simulink model "Parallel_Inverter_VSG"  (R2021b)
settings: Solver=FixedStepAuto  StartTime=0.0  StopTime=1  RelTol=1e-3
libraries: spsSeriesRLCBranchLib x11, spsCurrentMeasurementLib x4, spsVoltageMeasurementLib x4, spsDCVoltageSourceLib x2, powerlib_extras x2, spsTHDLib x2, spsUniversalBridgeLib x2, simulink x2, spspowerguiLib x1
settings Model: SimulationMode=accelerator  Creator=abc6820292  LastModifiedBy=abc6820292
settings SolverCC: ZeroCrossControl=EnableAll  ZeroCrossAlgorithm=Adaptive
settings SFSimCC: SimTargetLang=C++
settings RTWCC: BuildConfiguration=Faster Runs

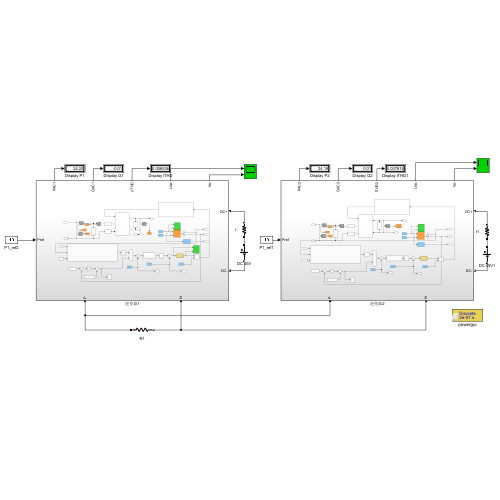
[thumbnail: Simulink's stored preview of the top-level diagram]
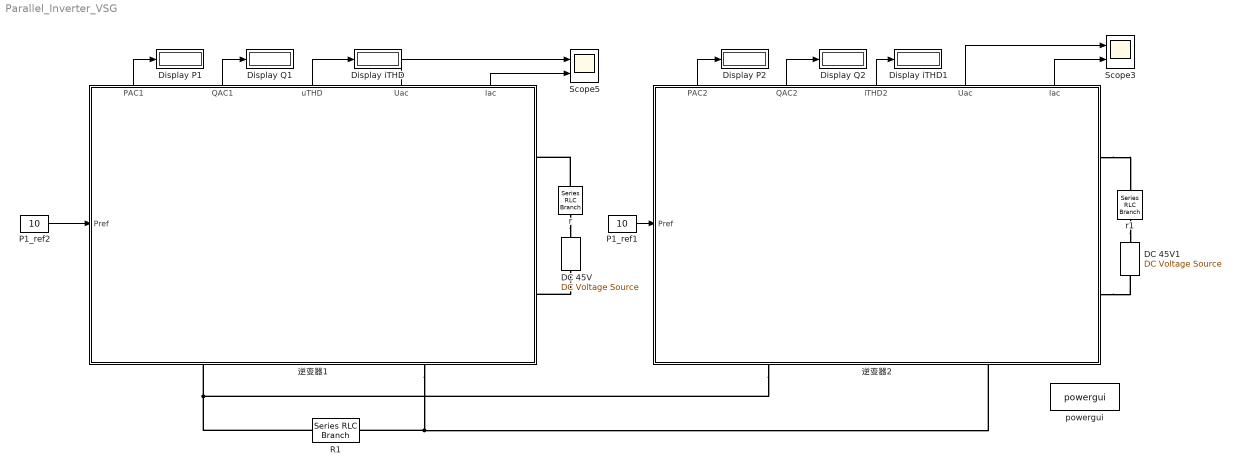
== system Parallel_Inverter_VSG ==
  DC 45V : spsDCVoltageSourceLib/DC Voltage Source  Amplitude=45  Measurements=None
  DC 45V1 : spsDCVoltageSourceLib/DC Voltage Source  Amplitude=45  Measurements=None
  Display P1 : Display
      settings: Format=bank
  Display P2 : Display
      settings: Format=bank
  Display Q1 : Display
      settings: Format=bank
  Display Q2 : Display
      settings: Format=bank
  Display iTHD : Display
  Display iTHD1 : Display
  P1_ref1 : Constant  Value=10
  P1_ref2 : Constant  Value=10
  R1 : spsSeriesRLCBranchLib/Series RLC Branch  LConnTagsString=__new0  RConnTagsString=__new0  BranchType=R  Resistance=12  Inductance=0  SetiL0=off  InitialCurrent=0  Capacitance=3e-4  Setx0=off  InitialVoltage=350  Measurements=None
  Scope3 : Scope  NumInputPorts=2
  Scope5 : Scope  NumInputPorts=2
  powergui : spspowerguiLib/powergui  SimulationMode=Discrete  SampleTime=2e-7  frequency=60  Iterations=50  frequencyindice=0  Pbase=100e6  ErrMax=1e-4  UnitsV=kV  UnitsW=MW  buscounter=0  FunctionMessages=off  echomessages=off  EnableUseOfTLC=off  CurrentSourceSwitches=off  DisableSnubberDevices=off  DisableRonSwitches=off  DisableVfSwitches=off  DisplayEquations=off  AutomaticDiscreteSolvers=off  SolverType=Tustin/Backward Euler (TBE)  Interpol=off  ExternalGateDelay=off  methode=off  Ts=0  x0status=blocks  SPID=off  SwTol=0  HookPort=off  NonlinearTolerance=1e-4  nMaxIteration=100  ContinueOnMaxIteration=off  RestoreLinks=warning  ResistiveCurrentMeasurement=off  Frange=[0:2:500]  Ylog=off  Xlog=on  ShowGrid=off  save=off  variable=ZData  structure=QQQQQ  ZoomFFT=off  StartTime=0.5  cycles=15  DisplayStyle=1  fundamental=50  FreqAxis=off  MaxFrequency=1000  frequencyindicesteady=1  RmsSteady=1  display=off
  r : spsSeriesRLCBranchLib/Series RLC Branch  LConnTagsString=__new0  RConnTagsString=__new0  BranchType=R  Resistance=0.05  Inductance=0  SetiL0=off  InitialCurrent=0  Capacitance=2e-3  Setx0=on  InitialVoltage=390  Measurements=None
  r1 : spsSeriesRLCBranchLib/Series RLC Branch  LConnTagsString=__new0  RConnTagsString=__new0  BranchType=R  Resistance=0.05  Inductance=0  SetiL0=off  InitialCurrent=0  Capacitance=2e-3  Setx0=on  InitialVoltage=390  Measurements=None
  逆变器1 : Subsystem
      settings: PortSchema="{\"entries\":[{\"content\":{\"sides\":[{\"content\":{\"connectorIds\":[\"In1\"]},\"type\":\"ConnectorPlacement.EquallySpacedRectSide\",\"uuid\":\"bea3d649-ea16-4ede-b4a3-db27428ff183\"},{\"content\":{\"connectorIds\":[\"RConn1\",\"RConn2\"],\"side\":\"RIGHT\"},\"type\":\"ConnectorPlacement.EquallySpacedRectSide\",\"uuid\":\"c4ad4349-eb8f-48f4-b2b9-d35e08430d05\"},{\"content\":{\"connectorIds\":[\"Out1\",\"Out2\",\"Out3\",\"Out4\",\"Out5\"],\"side\":\"TOP\"},\"type\":\"ConnectorPlacement.EquallySpacedRectSide\",\"uuid\":\"7c68d96b-b93d-4a12-819a-4c9a93b50c2f\"},{\"content\":{\"connectorIds\":[\"RConn3\",\"RConn4\"],\"side\":\"BOTTOM\"},\"type\":\"ConnectorPlacement.EquallySpacedRectSide\",\"uuid\":\"1109a0f2-0200-4778-be81-be65e9d67cf4\"}]},\"type\":\"ConnectorPlacement.EquallySpacedConnector\",\"uuid\":\"8557925e-2abb-4538-b581-1ff4712c6dfe\"}],\"packageUris\":[\"http://schema.mathworks.com/mf0/Connector/R2020b\"],\"version\":\"1.0\"}"
  逆变器2 : Subsystem
      settings: PortSchema="{\"entries\":[{\"content\":{\"sides\":[{\"content\":{\"connectorIds\":[\"In1\"]},\"type\":\"ConnectorPlacement.EquallySpacedRectSide\",\"uuid\":\"bea3d649-ea16-4ede-b4a3-db27428ff183\"},{\"content\":{\"connectorIds\":[\"RConn1\",\"RConn2\"],\"side\":\"RIGHT\"},\"type\":\"ConnectorPlacement.EquallySpacedRectSide\",\"uuid\":\"c4ad4349-eb8f-48f4-b2b9-d35e08430d05\"},{\"content\":{\"connectorIds\":[\"Out1\",\"Out2\",\"Out3\",\"Out4\",\"Out5\"],\"side\":\"TOP\"},\"type\":\"ConnectorPlacement.EquallySpacedRectSide\",\"uuid\":\"7c68d96b-b93d-4a12-819a-4c9a93b50c2f\"},{\"content\":{\"connectorIds\":[\"RConn3\",\"RConn4\"],\"side\":\"BOTTOM\"},\"type\":\"ConnectorPlacement.EquallySpacedRectSide\",\"uuid\":\"1109a0f2-0200-4778-be81-be65e9d67cf4\"}]},\"type\":\"ConnectorPlacement.EquallySpacedConnector\",\"uuid\":\"8557925e-2abb-4538-b581-1ff4712c6dfe\"}],\"packageUris\":[\"http://schema.mathworks.com/mf0/Connector/R2020b\"],\"version\":\"1.0\"}"
  wires:
  逆变器1/1(PAC1) -> Display P1/1
  逆变器1/2(QAC1) -> Display Q1/1
  逆变器1/3(uTHD) -> Display iTHD/1
  逆变器2/5(Iac) -> Scope3/2
  逆变器2/4(Uac) -> Scope3/1
  逆变器2/3(iTHD2) -> Display iTHD1/1
  P1_ref2/1 -> 逆变器1/1(Pref)
  P1_ref1/1 -> 逆变器2/1(Pref)
  逆变器2/2(QAC2) -> Display Q2/1
  逆变器2/1(PAC2) -> Display P2/1
  逆变器1/4(Uac) -> Scope5/1
  逆变器1/5(Iac) -> Scope5/2
  connections:
  DC 45V/LConn1 -- 逆变器1/RConn2
  r/RConn1 -- DC 45V/RConn1
  r/LConn1 -- 逆变器1/RConn1
  逆变器2/RConn2 -- DC 45V1/LConn1
  逆变器2/RConn1 -- r1/LConn1
  r1/RConn1 -- DC 45V1/RConn1
  逆变器2/RConn3 -- R1/LConn1 -- 逆变器1/RConn3
  逆变器1/RConn4 -- 逆变器2/RConn4 -- R1/RConn1

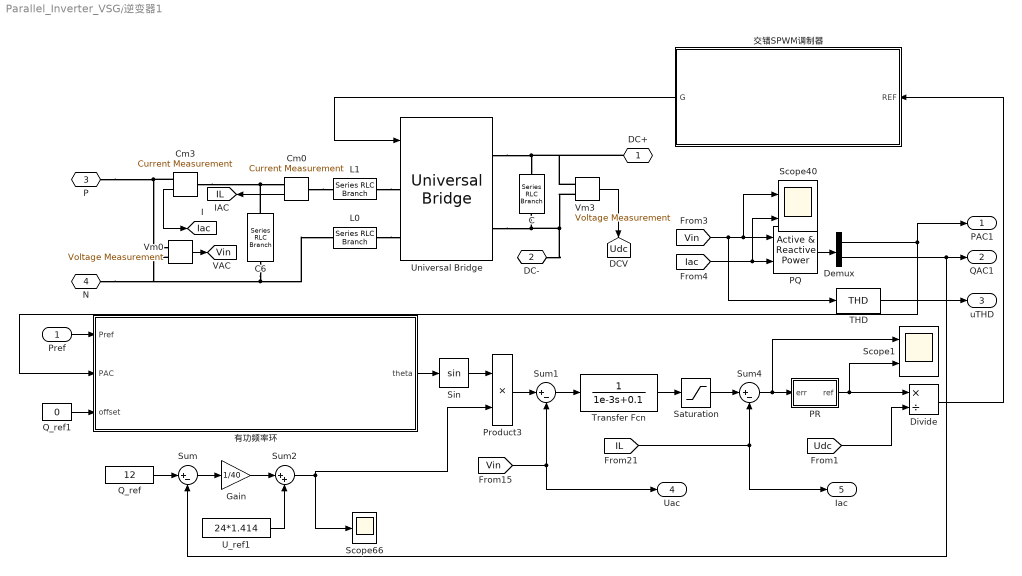
== system Parallel_Inverter_VSG/逆变器1 ==
  Pref : Inport
  C : spsSeriesRLCBranchLib/Series RLC Branch  LConnTagsString=__new0  RConnTagsString=__new0  BranchType=C  Resistance=0.05  Inductance=0  SetiL0=off  InitialCurrent=0  Capacitance=4e-3  Setx0=on  InitialVoltage=45  Measurements=None
  C6 : spsSeriesRLCBranchLib/Series RLC Branch  LConnTagsString=__new0  RConnTagsString=__new0  BranchType=RC  Resistance=1  Inductance=0  SetiL0=off  InitialCurrent=0  Capacitance=3e-6  Setx0=off  InitialVoltage=350  Measurements=None
  Cm0 : spsCurrentMeasurementLib/Current Measurement  PhasorSimulation=off  OutputType=Complex  PSBequivalent=0
  Cm3 : spsCurrentMeasurementLib/Current Measurement  PhasorSimulation=off  OutputType=Complex  PSBequivalent=0
  Demux : Demux  Outputs=2
  Divide : Product  Inputs=*/
  Gain : Gain  Gain=1/40
  L0 : spsSeriesRLCBranchLib/Series RLC Branch  LConnTagsString=__new0  RConnTagsString=__new0  BranchType=RL  Resistance=81e-3  Inductance=5e-4  SetiL0=off  InitialCurrent=0  Capacitance=inf  Setx0=off  InitialVoltage=0  Measurements=None
  L1 : spsSeriesRLCBranchLib/Series RLC Branch  LConnTagsString=__new0  RConnTagsString=__new0  BranchType=RL  Resistance=81e-3  Inductance=5e-4  SetiL0=off  InitialCurrent=0  Capacitance=inf  Setx0=off  InitialVoltage=0  Measurements=None
  PQ : powerlib_extras/Measurements/Active & Reactive Power  f1=50
      settings: SourceProductBaseCode=PS
  PR : Subsystem  TreatAsAtomicUnit=on  mask{Kp=4, Kr=100, Wc=5, Upper=100, Lower=-100}
  Product3 : Product
  Q_ref : Constant  Value=12
  Q_ref1 : Constant  Value=0
  Saturation : Saturate  UpperLimit=30  LowerLimit=-30
  Scope1 : Scope  NumInputPorts=2
  Scope40 : Scope  NumInputPorts=2
  Scope66 : Scope
  Sin : Trigonometry
  Sum : Sum  Inputs=|+-
  Sum1 : Sum  Inputs=|+-
  Sum2 : Sum  Inputs=|++
  Sum4 : Sum  Inputs=|+-
  THD : spsTHDLib/THD  Freq=50  Ts=0
      settings: SourceProductBaseCode=PS
  Transfer Fcn : TransferFcn  Denominator=[1e-3 0.1]
  U_ref1 : Constant  Value=24*1.414
  Universal Bridge : spsUniversalBridgeLib/Universal Bridge  Arms=2  SnubberResistance=1e5  SnubberCapacitance=inf  Device=MOSFET / Diodes  Ron=0.01  Lon=0  ForwardVoltages="[  0  0  ]"  ForwardVoltage=0  GTOparameters=[ 10e-6 , 20e-6 ]  IGBTparameters=[ 1e-6 , 2e-6 ]  Measurements=None  Measurements_2=None  converterType=Rectifier
  Vm0 : spsVoltageMeasurementLib/Voltage Measurement  PhasorSimulation=off  OutputType=Complex  PSBequivalent=0
  Vm3 : spsVoltageMeasurementLib/Voltage Measurement  PhasorSimulation=off  OutputType=Complex  PSBequivalent=0
  交错SPWM调制器 : Subsystem
  有功频率环 : Subsystem
  DC+ : PMIOPort  Side=Right
  DC- : PMIOPort  Port=2  Side=Right
  P : PMIOPort  Port=3  Side=Right
  N : PMIOPort  Port=4  Side=Right
  PAC1 : Outport
  QAC1 : Outport  Port=2
  uTHD : Outport  Port=3
  Uac : Outport  Port=4
  Iac : Outport  Port=5
  tag scope: IL=global, Iac=global, Udc=global, Vin=global
  wires:
  Vm0/1 -> [Vin]
  Cm0/1 -> [IL]
  Vm3/1 -> [Udc]
  Cm3/1 -> [Iac]
  Sum/1 -> Gain/1
  Saturation/1 -> Sum4/1
  Sum4/1 -> Scope1/1, PR/1(err)
  Pref/1 -> 有功频率环/1(Pref)
  有功频率环/1(theta) -> Sin/1
  PR/1(ref) -> Divide/1, Scope1/2
  Gain/1 -> Sum2/1
  Divide/1 -> 交错SPWM调制器/1(REF)
  [Udc] -> Divide/2
  Sum2/1 -> Product3/2, Scope66/1
  Sin/1 -> Product3/1
  Product3/1 -> Sum1/1
  Q_ref/1 -> Sum/1
  U_ref1/1 -> Sum2/2
  [Vin] -> Uac/1, Sum1/2
  [IL] -> Iac/1, Sum4/2
  交错SPWM调制器/1(G) -> Universal Bridge/1
  THD/1 -> uTHD/1
  Demux/2 -> QAC1/1, Sum/2
  [Iac] -> Scope40/2, PQ/2
  PQ/1 -> Demux/1
  Demux/1 -> PAC1/1, 有功频率环/2(PAC)
  Q_ref1/1 -> 有功频率环/3(offset)
  Sum1/1 -> Transfer Fcn/1
  Transfer Fcn/1 -> Saturation/1
  [Vin] -> Scope40/1, PQ/1, THD/1
  connections:
  L0/LConn1 -- Universal Bridge/LConn2
  Vm3/LConn2 -- DC-/RConn1 -- C/RConn1 -- Universal Bridge/RConn2
  L1/LConn1 -- Universal Bridge/LConn1
  C6/LConn1 -- Cm3/LConn1 -- Cm0/RConn1
  Cm0/LConn1 -- L1/RConn1
  C6/RConn1 -- N/RConn1 -- Vm0/LConn2 -- L0/RConn1
  Universal Bridge/RConn1 -- DC+/RConn1 -- Vm3/LConn1 -- C/LConn1
  Cm3/RConn1 -- P/RConn1 -- Vm0/LConn1

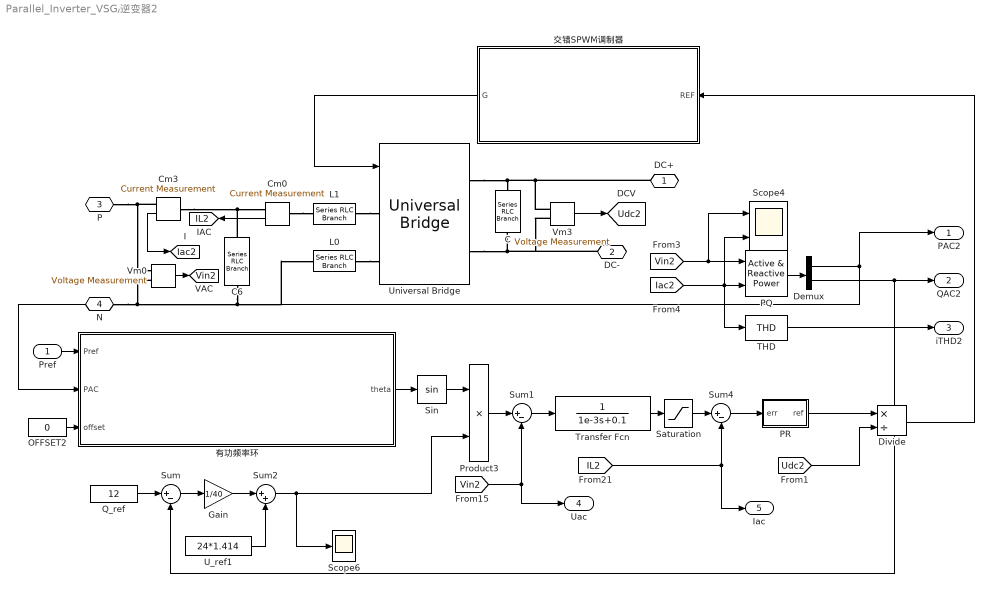
== system Parallel_Inverter_VSG/逆变器2 ==
  Pref : Inport
  C : spsSeriesRLCBranchLib/Series RLC Branch  LConnTagsString=__new0  RConnTagsString=__new0  BranchType=C  Resistance=0.05  Inductance=0  SetiL0=off  InitialCurrent=0  Capacitance=3e-3  Setx0=on  InitialVoltage=45  Measurements=None
  C6 : spsSeriesRLCBranchLib/Series RLC Branch  LConnTagsString=__new0  RConnTagsString=__new0  BranchType=RC  Resistance=1  Inductance=0  SetiL0=off  InitialCurrent=0  Capacitance=3e-6  Setx0=off  InitialVoltage=350  Measurements=None
  Cm0 : spsCurrentMeasurementLib/Current Measurement  PhasorSimulation=off  OutputType=Complex  PSBequivalent=0
  Cm3 : spsCurrentMeasurementLib/Current Measurement  PhasorSimulation=off  OutputType=Complex  PSBequivalent=0
  Demux : Demux  Outputs=2
  Divide : Product  Inputs=*/
  Gain : Gain  Gain=1/40
  L0 : spsSeriesRLCBranchLib/Series RLC Branch  LConnTagsString=__new0  RConnTagsString=__new0  BranchType=RL  Resistance=0.05  Inductance=5e-4  SetiL0=off  InitialCurrent=0  Capacitance=inf  Setx0=off  InitialVoltage=0  Measurements=None
  L1 : spsSeriesRLCBranchLib/Series RLC Branch  LConnTagsString=__new0  RConnTagsString=__new0  BranchType=RL  Resistance=0.05  Inductance=5e-4  SetiL0=off  InitialCurrent=0  Capacitance=inf  Setx0=off  InitialVoltage=0  Measurements=None
  OFFSET2 : Constant  Value=0
  PQ : powerlib_extras/Measurements/Active & Reactive Power  f1=50
      settings: SourceProductBaseCode=PS
  PR : Subsystem  TreatAsAtomicUnit=on  mask{Kp=4, Kr=100, Wc=5, Upper=100, Lower=-100}
  Product3 : Product
  Q_ref : Constant  Value=12
  Saturation : Saturate  UpperLimit=30  LowerLimit=-30
  Scope4 : Scope  NumInputPorts=2
  Scope6 : Scope
  Sin : Trigonometry
  Sum : Sum  Inputs=|+-
  Sum1 : Sum  Inputs=|+-
  Sum2 : Sum  Inputs=|++
  Sum4 : Sum  Inputs=|+-
  THD : spsTHDLib/THD  Freq=50  Ts=0
      settings: SourceProductBaseCode=PS
  Transfer Fcn : TransferFcn  Denominator=[1e-3 0.1]
  U_ref1 : Constant  Value=24*1.414
  Universal Bridge : spsUniversalBridgeLib/Universal Bridge  Arms=2  SnubberResistance=1e5  SnubberCapacitance=inf  Device=MOSFET / Diodes  Ron=1e-2  Lon=0  ForwardVoltages="[  0  0  ]"  ForwardVoltage=0  GTOparameters=[ 10e-6 , 20e-6 ]  IGBTparameters=[ 1e-6 , 2e-6 ]  Measurements=None  Measurements_2=None  converterType=Rectifier
  Vm0 : spsVoltageMeasurementLib/Voltage Measurement  PhasorSimulation=off  OutputType=Complex  PSBequivalent=0
  Vm3 : spsVoltageMeasurementLib/Voltage Measurement  PhasorSimulation=off  OutputType=Complex  PSBequivalent=0
  交错SPWM调制器 : Subsystem
  有功频率环 : Subsystem
  DC+ : PMIOPort  Side=Right
  DC- : PMIOPort  Port=2  Side=Right
  P : PMIOPort  Port=3  Side=Right
  N : PMIOPort  Port=4  Side=Right
  PAC2 : Outport
  QAC2 : Outport  Port=2
  iTHD2 : Outport  Port=3
  Uac : Outport  Port=4
  Iac : Outport  Port=5
  tag scope: IL2=global, Iac2=global, Udc2=global, Vin2=global
  wires:
  Vm0/1 -> [Vin2]
  Cm0/1 -> [IL2]
  Vm3/1 -> [Udc2]
  Cm3/1 -> [Iac2]
  Sum/1 -> Gain/1
  Saturation/1 -> Sum4/1
  Sum4/1 -> PR/1(err)
  Pref/1 -> 有功频率环/1(Pref)
  有功频率环/1(theta) -> Sin/1
  PR/1(ref) -> Divide/1
  Gain/1 -> Sum2/1
  Divide/1 -> 交错SPWM调制器/1(REF)
  [Udc2] -> Divide/2
  Sum2/1 -> Product3/2, Scope6/1
  Sin/1 -> Product3/1
  Product3/1 -> Sum1/1
  Q_ref/1 -> Sum/1
  U_ref1/1 -> Sum2/2
  [Vin2] -> Uac/1, Sum1/2
  [IL2] -> Iac/1, Sum4/2
  交错SPWM调制器/1(G) -> Universal Bridge/1
  THD/1 -> iTHD2/1
  Demux/2 -> QAC2/1, Sum/2
  [Iac2] -> THD/1, Scope4/2, PQ/2
  PQ/1 -> Demux/1
  Demux/1 -> PAC2/1, 有功频率环/2(PAC)
  [Vin2] -> Scope4/1, PQ/1
  OFFSET2/1 -> 有功频率环/3(offset)
  Sum1/1 -> Transfer Fcn/1
  Transfer Fcn/1 -> Saturation/1
  connections:
  L0/LConn1 -- Universal Bridge/LConn2
  Universal Bridge/RConn2 -- DC-/RConn1 -- Vm3/LConn2 -- C/RConn1
  L1/LConn1 -- Universal Bridge/LConn1
  C6/LConn1 -- Cm3/LConn1 -- Cm0/RConn1
  Cm0/LConn1 -- L1/RConn1
  Vm0/LConn2 -- C6/RConn1 -- L0/RConn1 -- N/RConn1
  Vm3/LConn1 -- DC+/RConn1 -- Universal Bridge/RConn1 -- C/LConn1
  Cm3/RConn1 -- P/RConn1 -- Vm0/LConn1

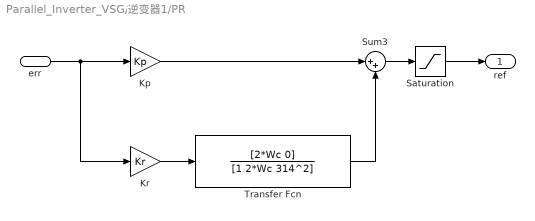
== system Parallel_Inverter_VSG/逆变器1/PR ==
  err : Inport
  Kp : Gain  Gain=Kp
  Kr : Gain  Gain=Kr
  Saturation : Saturate  UpperLimit=Upper  LowerLimit=Lower
  Sum3 : Sum  Inputs=|++
  Transfer Fcn : TransferFcn  Numerator=[2*Wc 0]  Denominator=[1 2*Wc 314^2]
  ref : Outport
  wires:
  Kp/1 -> Sum3/1
  Sum3/1 -> Saturation/1
  err/1 -> Kr/1, Kp/1
  Kr/1 -> Transfer Fcn/1
  Transfer Fcn/1 -> Sum3/2
  Saturation/1 -> ref/1

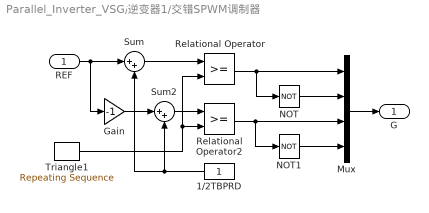
== system Parallel_Inverter_VSG/逆变器1/交错SPWM调制器 ==
  REF : Inport
  1/2TBPRD : Constant
  Gain : Gain  Gain=-1
  Mux : Mux
  NOT : Logic  Operator=NOT  IconShape=distinctive  AllPortsSameDT=off  OutDataTypeStr=boolean
  NOT1 : Logic  Operator=NOT  IconShape=distinctive  AllPortsSameDT=off  OutDataTypeStr=boolean
  Relational Operator : RelationalOperator  OutDataTypeStr=boolean  RndMeth=Nearest
  Relational Operator2 : RelationalOperator  OutDataTypeStr=boolean  RndMeth=Nearest
  Sum : Sum  Inputs=|++
  Sum2 : Sum  Inputs=|++
  Triangle1 : simulink/Sources/Repeating Sequence  rep_seq_t=[0 1/16000/2 1/16000]  rep_seq_y=[0 2 0]
  G : Outport
  wires:
  Triangle1/1 -> Relational Operator2/2, Relational Operator/2
  Sum/1 -> Relational Operator/1
  REF/1 -> Gain/1, Sum/1
  Gain/1 -> Sum2/1
  Sum2/1 -> Relational Operator2/1
  1/2TBPRD/1 -> Sum/2, Sum2/2
  Relational Operator/1 -> NOT/1, Mux/1
  NOT/1 -> Mux/2
  Mux/1 -> G/1
  NOT1/1 -> Mux/4
  Relational Operator2/1 -> NOT1/1, Mux/3

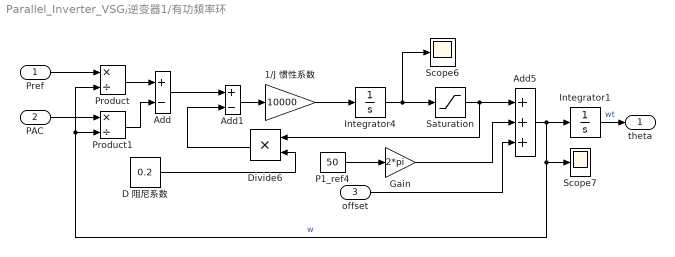
== system Parallel_Inverter_VSG/逆变器1/有功频率环 ==
  Pref : Inport
  PAC : Inport  Port=2
  offset : Inport  Port=3
  1/J 惯性系数 : Gain  Gain=10000
  Add : Sum  Inputs=+-
  Add1 : Sum  Inputs=+-
  Add5 : Sum  Inputs=+++
  D 阻尼系数 : Constant  Value=0.2
  Divide6 : Product  Inputs=**
  Gain : Gain  Gain=2*pi
  Integrator1 : Integrator  WrapState=on  WrappedStateUpperValue=2*pi  WrappedStateLowerValue=0
  Integrator4 : Integrator
  P1_ref4 : Constant  Value=50
  Product : Product  Inputs=*/
  Product1 : Product  Inputs=*/
  Saturation : Saturate  UpperLimit=15  LowerLimit=-10
  Scope6 : Scope
  Scope7 : Scope
  theta : Outport
  wires:
  Integrator4/1 -> Scope6/1, Saturation/1
  Integrator1/1 -> theta/1  "wt"
  Saturation/1 -> Add5/1, Divide6/1
  Add5/1 -> Integrator1/1, Scope7/1, Product/2, Product1/2  "w"
  Product1/1 -> Add/2
  Product/1 -> Add/1
  1/J 惯性系数/1 -> Integrator4/1
  Gain/1 -> Add5/2
  PAC/1 -> Product1/1
  Pref/1 -> Product/1
  Divide6/1 -> Add1/2
  D 阻尼系数/1 -> Divide6/2
  Add/1 -> Add1/1
  P1_ref4/1 -> Gain/1
  offset/1 -> Add5/3
  Add1/1 -> 1/J 惯性系数/1

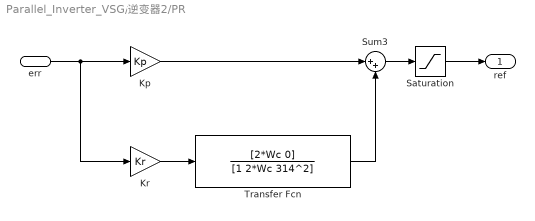
== system Parallel_Inverter_VSG/逆变器2/PR ==
  err : Inport
  Kp : Gain  Gain=Kp
  Kr : Gain  Gain=Kr
  Saturation : Saturate  UpperLimit=Upper  LowerLimit=Lower
  Sum3 : Sum  Inputs=|++
  Transfer Fcn : TransferFcn  Numerator=[2*Wc 0]  Denominator=[1 2*Wc 314^2]
  ref : Outport
  wires:
  Kp/1 -> Sum3/1
  Sum3/1 -> Saturation/1
  err/1 -> Kr/1, Kp/1
  Kr/1 -> Transfer Fcn/1
  Transfer Fcn/1 -> Sum3/2
  Saturation/1 -> ref/1

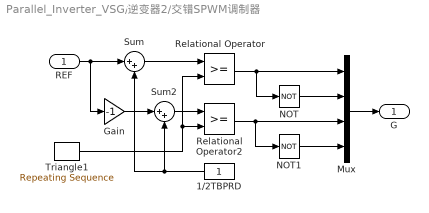
== system Parallel_Inverter_VSG/逆变器2/交错SPWM调制器 ==
  REF : Inport
  1/2TBPRD : Constant
  Gain : Gain  Gain=-1
  Mux : Mux
  NOT : Logic  Operator=NOT  IconShape=distinctive  AllPortsSameDT=off  OutDataTypeStr=boolean
  NOT1 : Logic  Operator=NOT  IconShape=distinctive  AllPortsSameDT=off  OutDataTypeStr=boolean
  Relational Operator : RelationalOperator  OutDataTypeStr=boolean  RndMeth=Nearest
  Relational Operator2 : RelationalOperator  OutDataTypeStr=boolean  RndMeth=Nearest
  Sum : Sum  Inputs=|++
  Sum2 : Sum  Inputs=|++
  Triangle1 : simulink/Sources/Repeating Sequence  rep_seq_t=[0 1/16000/2 1/16000]  rep_seq_y=[2 0 2]
  G : Outport
  wires:
  Triangle1/1 -> Relational Operator2/2, Relational Operator/2
  Sum/1 -> Relational Operator/1
  REF/1 -> Gain/1, Sum/1
  Gain/1 -> Sum2/1
  Sum2/1 -> Relational Operator2/1
  1/2TBPRD/1 -> Sum/2, Sum2/2
  Relational Operator/1 -> NOT/1, Mux/1
  NOT/1 -> Mux/2
  Mux/1 -> G/1
  NOT1/1 -> Mux/4
  Relational Operator2/1 -> NOT1/1, Mux/3

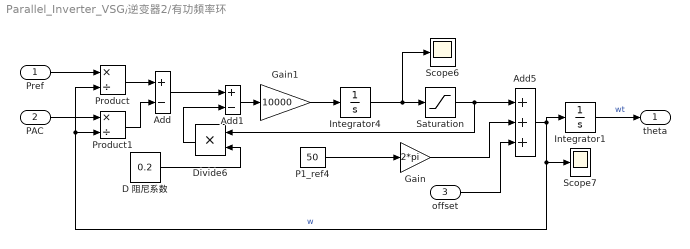
== system Parallel_Inverter_VSG/逆变器2/有功频率环 ==
  Pref : Inport
  PAC : Inport  Port=2
  offset : Inport  Port=3
  Add : Sum  Inputs=+-
  Add1 : Sum  Inputs=+-
  Add5 : Sum  Inputs=+++
  D 阻尼系数 : Constant  Value=0.2
  Divide6 : Product  Inputs=**
  Gain : Gain  Gain=2*pi
  Gain1 : Gain  Gain=10000
  Integrator1 : Integrator  WrapState=on  WrappedStateUpperValue=2*pi  WrappedStateLowerValue=0
  Integrator4 : Integrator
  P1_ref4 : Constant  Value=50
  Product : Product  Inputs=*/
  Product1 : Product  Inputs=*/
  Saturation : Saturate  UpperLimit=15  LowerLimit=-10
  Scope6 : Scope
  Scope7 : Scope
  theta : Outport
  wires:
  Integrator4/1 -> Scope6/1, Saturation/1
  Integrator1/1 -> theta/1  "wt"
  Saturation/1 -> Add5/1, Divide6/1
  Add5/1 -> Integrator1/1, Scope7/1, Product/2, Product1/2  "w"
  Product1/1 -> Add/2
  Product/1 -> Add/1
  Gain/1 -> Add5/2
  PAC/1 -> Product1/1
  Pref/1 -> Product/1
  Divide6/1 -> Add1/2
  D 阻尼系数/1 -> Divide6/2
  Add/1 -> Add1/1
  P1_ref4/1 -> Gain/1
  offset/1 -> Add5/3
  Add1/1 -> Gain1/1
  Gain1/1 -> Integrator4/1
